simulink model "diff_equ"  (R2026a)
settings: Solver=VariableStepAuto  StopTime=0.02
settings Model: Creator=HAKAN SARI  LastModifiedBy=HAKAN SARI

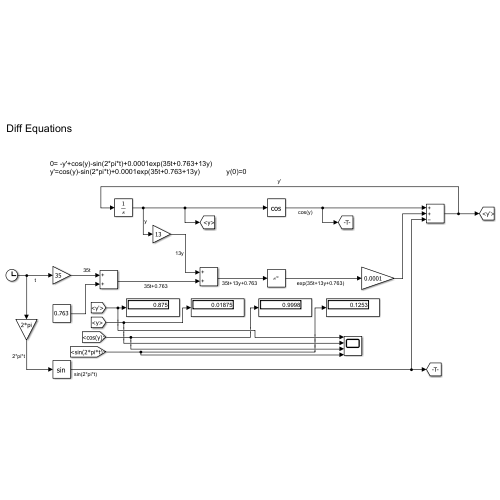
[thumbnail: Simulink's stored preview of the top-level diagram]
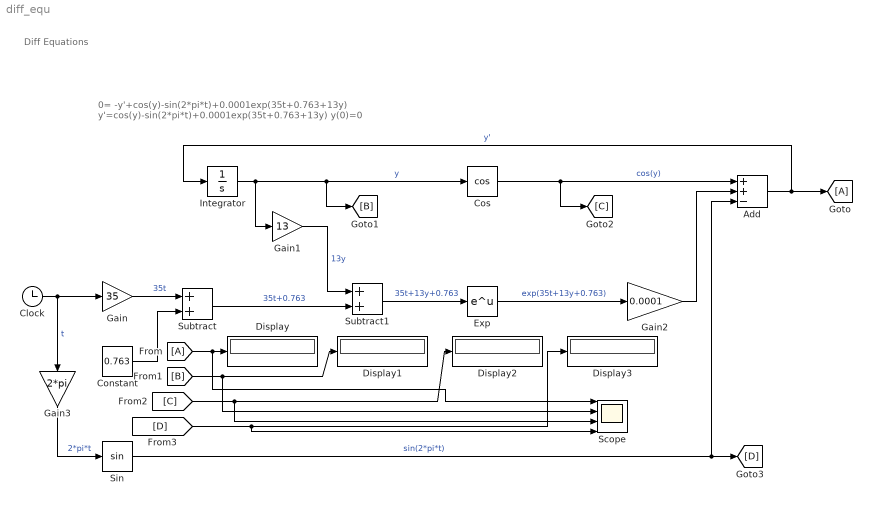
== system diff_equ ==
  note: Diff Equations
  note: 0= -y'+cos(y)-sin(2*pi*t)+0.0001exp(35t+0.763+13y)
      | y'=cos(y)-sin(2*pi*t)+0.0001exp(35t+0.763+13y) y(0)=0
  Add : Sum  Inputs=++-
  Clock : Clock
  Constant : Constant  Value=0.763
  Cos : Trigonometry  Operator=cos
  Display{,1..3} (4 alike) : Display
  Exp : Math
  From : From
  Gain : Gain  Gain=35
  Gain1 : Gain  Gain=13
  Gain2 : Gain  Gain=0.0001
  Gain3 : Gain  Gain=2*pi
  Goto : Goto
  Integrator : Integrator
  Scope : Scope  NumInputPorts=4
      settings: ActiveDisplayYMinimum=0.85939553281473469  ActiveDisplayYMaximum=1.0158610186518107
  Sin : Trigonometry
  Subtract : Sum
  Subtract1 : Sum
  wires:
  Integrator/1 -> [B], Cos/1, Gain1/1  "y"
  Add/1 -> Integrator/1, Goto/1  "y'"
  Clock/1 -> Gain/1, Gain3/1  "t"
  Gain/1 -> Subtract/1  "35t"
  Constant/1 -> Subtract/2
  Subtract/1 -> Subtract1/2  "35t+0.763"
  Exp/1 -> Gain2/1  "exp(35t+13y+0.763)"
  Subtract1/1 -> Exp/1  "35t+13y+0.763"
  Gain1/1 -> Subtract1/1  "13y"
  Sin/1 -> [D], Add/3  "sin(2*pi*t)"
  Gain3/1 -> Sin/1  "2*pi*t"
  Cos/1 -> [C], Add/1  "cos(y)"
  Gain2/1 -> Add/2
  From/1 -> Scope/1, Display/1
  [B] -> Scope/2, Display1/1
  [C] -> Scope/3, Display2/1
  [D] -> Scope/4, Display3/1
